simulink model "USV_SAR_MovingTarget"  (R2026b)
settings: Solver=VariableStepAuto  StopTime=600
undefined symbols (not defined in the file): arrival_dwell_time, arrival_radius, arrival_speed, assistance_duration, current_bias_x, current_bias_y, current_change_time, current_estimation_tau, current_x, drag_r, drag_u, F_max, home_x, home_y, inertia_z, initial_heading, initial_x, initial_y, integral_activation_radius, K_aw, K_distance, Kd_heading, Ki_position, Ki_u, Kp_heading, Kp_u, M_max, mass_usv, num_waypoints, position_integral_limit, sar_detection_range, sar_drift_factor, sar_target_x, sar_target_y, u_max, waypoints
libraries: simulink x6
settings Model: Creator=pablo  LastModifiedBy=pablo

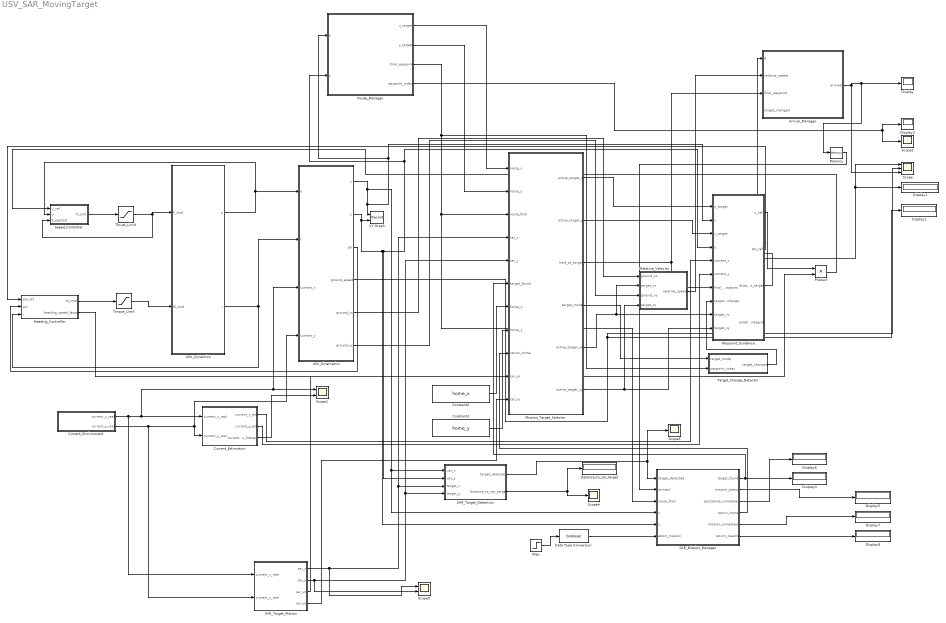
== system USV_SAR_MovingTarget ==
  Arrival_Manager : Stateflow chart  TreatAsAtomicUnit=on
  Constant2 : Constant  Value=home_x
  Constant3 : Constant  Value=home_y
  Current_Environment : Subsystem
  Current_Estimation : Subsystem
  Data Type Conversion : DataTypeConversion  OutDataTypeStr=boolean  SaturateOnIntegerOverflow=off  RndMeth=Floor
  Display{,1..8} (9 alike) : Display
  Heading_Controller : Subsystem
  Memory : Memory
  Mission_Target_Selector : Subsystem
  Product : Product
  Relative_Velocity : Subsystem
  Route_Manager : Stateflow chart  TreatAsAtomicUnit=on
  SAR_Mission_Manager : Stateflow chart  TreatAsAtomicUnit=on
  SAR_Target_Detection : Subsystem
  SAR_Target_Motion : Subsystem
  Scope : Scope  NumInputPorts=3
      settings: ActiveDisplayYMinimum=-3.9141031212329302  ActiveDisplayYMaximum=39.009126348576444
  Scope1 : Scope  NumInputPorts=2
      settings: ActiveDisplayYMinimum=-0.25  ActiveDisplayYMaximum=0.25
  Scope2 : Scope
      settings: ActiveDisplayYMinimum=-8.8280515458215767  ActiveDisplayYMaximum=9.3125380233394175  DataLoggingVariableName=ScopeData2
  Scope3 : Scope
      settings: ActiveDisplayYMinimum=0.096949603045415472  ActiveDisplayYMaximum=1.0318774717483707  DataLoggingVariableName=ScopeData3
  Scope4 : Scope
      settings: ActiveDisplayYMinimum=-1.9004946435428702E+6  ActiveDisplayYMaximum=1.5322246928084393E+6  DataLoggingVariableName=ScopeData4
  Scope5 : Scope  NumInputPorts=2
      settings: ActiveDisplayYMinimum=-44.000000000000014  ActiveDisplayYMaximum=76.000000000000028  DataLoggingVariableName=ScopeData5
  Speed_Controller : Subsystem
  Step : Step  Time=100  FinalValue=0  SampleTime=0
  Target_Change_Detector : Subsystem
  Thrust_Limit : Saturate  UpperLimit=F_max  LowerLimit=-F_max
  Torque_Limit : Saturate  UpperLimit=M_max  LowerLimit=-M_max
  USV_Dynamics : Subsystem
  USV_Kinematics : Subsystem
  Waypoint_Guidance : Subsystem
  XY Graph : Record  NumPorts=2.0  FileSettingsInternal="{\"entries\":[{\"content\":{\"excelSettings\":{\"content\":{},\"type\":\"Streamout.ExcelSettings\"},\"parquetSettings\":{\"content\":{},\"type\":\"Streamout.ParquetSettings\"}},\"type\":\"Streamout.FileSettingStorage\",\"uuid\":\"\"}],\"packageUris\":[\"http:\\/\\/schema.mathworks.com\\/mf0\\/streamout_blocks\\/R2020a\"],\"version\":\"1.0\"}"  FrameSettings=[0, 0]  Layout=[1 1]  SignalsInternal="{\"entries\":[{\"content\":{\"signals\":[{\"content\":{\"blockPath\":[],\"dimensions\":[1],\"domain\":\"\",\"lineColor\":\"#a2142f\",\"plots\":[ 1 ],\"port\":1,\"sid\":[\"\"],\"signalID\":1,\"signalName\":\"USV_Kinematics:1\"},\"type\":\"RecordBlkView.Signal\",\"uuid\":\"\"},{\"content\":{\"blockPath\":[],\"dimensions\":[1],\"domain\":\"\",\"lineColor\":\"#139fff\",\"plots\":[ 1 ],\"port\":2,\"sid\":[\"\"],\"signalID\":2,\"signalName\":\"USV_Kinematics:2\"},\"type\":\"RecordBlkView.Signal\",\"uuid\":\"\"}]},\"type\":\"RecordBlkView.InputSignals\",\"uuid\":\"\"}],\"packageUris\":[\"http:\\/\\/schema.mathworks.com\\/mf0\\/streamout_blocks\\/R2020a\"],\"version\":\"1.0\"}"  VisualizationBindings="{\"xyplotplugin\":{\"info\":[{\"series\":[{\"bindingParametersList\":[{\"parameter\":\"X-Axis\",\"signalID\":1,\"signalName\":\"USV_Kinematics:1\"},{\"parameter\":\"Y-Axis\",\"signalID\":2,\"signalName\":\"USV_Kinematics:2\"}],\"seriesID\":0},{\"bindingParametersList\":[],\"seriesID\":1}],\"subplotID\":1}]}}"  CompatibilityTag=XY
  distance_to_sar_target : Display
  wires:
  USV_Dynamics/1(u) -> Speed_Controller/2(u), USV_Kinematics/1(u)
  USV_Dynamics/2(r) -> Heading_Controller/3(r), USV_Kinematics/2(r)
  Speed_Controller/1(F_cmd) -> Thrust_Limit/1
  Heading_Controller/1(M_cmd) -> Torque_Limit/1
  USV_Kinematics/3(psi) -> Heading_Controller/2(psi)
  USV_Kinematics/1(x) -> SAR_Mission_Manager/4(x), SAR_Target_Detection/1(usv_x), XY Graph/1, Route_Manager/1(x), Waypoint_Guidance/2(x)
  USV_Kinematics/2(y) -> SAR_Mission_Manager/5(y), SAR_Target_Detection/2(usv_y), Route_Manager/2(y), Waypoint_Guidance/4(y), XY Graph/2
  Waypoint_Guidance/2(psi_ref) -> Heading_Controller/1(psi_ref)
  Waypoint_Guidance/1(u_ref) -> Product/1
  Arrival_Manager/1(arrived) -> Memory/1, Display/1, Scope/3
  Waypoint_Guidance/3(distance_to_target) -> Arrival_Manager/1(d), Scope/1, Display1/1
  Thrust_Limit/1 -> USV_Dynamics/1(F_cmd), Speed_Controller/3(F_applied)
  Torque_Limit/1 -> USV_Dynamics/2(M_cmd)
  Heading_Controller/2(heading_speed_factor) -> Product/2
  Product/1 -> Speed_Controller/1(u_ref)
  USV_Kinematics/4(ground_speed) -> Scope/2, Display2/1
  Current_Estimation/1(current_x_est) -> Waypoint_Guidance/5(current_x)
  Current_Estimation/2(current_y_est) -> Waypoint_Guidance/6(current_y)
  Current_Estimation/3(current_x_filtered) -> Scope1/2
  Current_Environment/1(current_x_real) -> SAR_Target_Motion/1(current_x_real), Scope1/1, USV_Kinematics/3(current_x), Current_Estimation/1(current_x_real)
  Current_Environment/2(current_y_real) -> SAR_Target_Motion/2(current_y_real), Current_Estimation/2(current_y_real), USV_Kinematics/4(current_y)
  Route_Manager/4(waypoint_index) -> Scope2/1, Display3/1
  SAR_Target_Motion/1(sar_x) -> Mission_Target_Selector/4(sar_x), SAR_Target_Detection/3(target_x), Scope5/1
  SAR_Target_Motion/2(sar_y) -> Mission_Target_Selector/5(sar_y), SAR_Target_Detection/4(target_y), Scope5/2
  SAR_Mission_Manager/1(target_found) -> Mission_Target_Selector/6(target_found), Display4/1
  SAR_Mission_Manager/2(mission_status) -> Display5/1
  Memory/1 -> SAR_Mission_Manager/2(arrived)
  SAR_Target_Detection/1(target_detected) -> Scope3/1, SAR_Mission_Manager/1(target_detected)
  SAR_Target_Detection/2(distance_to_sar_target) -> distance_to_sar_target/1, Scope4/1
  Mission_Target_Selector/3(hold_at_target) -> Arrival_Manager/3(final_waypoint), Waypoint_Guidance/7(final_waypoint)
  Route_Manager/1(x_target) -> Mission_Target_Selector/1(route_x)
  Route_Manager/2(y_target) -> Mission_Target_Selector/2(route_y)
  Route_Manager/3(final_waypoint) -> Target_Change_Detector/2(waypoint_index), SAR_Mission_Manager/3(route_final), Mission_Target_Selector/3(route_final)
  Mission_Target_Selector/1(active_target_x) -> Waypoint_Guidance/1(x_target)
  Mission_Target_Selector/2(active_target_y) -> Waypoint_Guidance/3(y_target)
  SAR_Mission_Manager/3(assistance_completed) -> Display6/1
  Constant2/1 -> Mission_Target_Selector/7(home_x)
  Constant3/1 -> Mission_Target_Selector/8(home_y)
  SAR_Mission_Manager/4(return_home) -> Mission_Target_Selector/9(return_home)
  SAR_Mission_Manager/5(mission_completed) -> Display7/1
  Step/1 -> Data Type Conversion/1
  Data Type Conversion/1 -> SAR_Mission_Manager/6(abort_mission)
  SAR_Mission_Manager/6(return_reason) -> Display8/1
  Target_Change_Detector/1(target_changed) -> Waypoint_Guidance/8(target_change)
  Mission_Target_Selector/4(target_mode) -> Target_Change_Detector/1(target_mode)
  SAR_Target_Motion/3(sar_vx) -> Mission_Target_Selector/10(sar_vx)
  SAR_Target_Motion/4(sar_vy) -> Mission_Target_Selector/11(sar_vy)
  Mission_Target_Selector/5(active_target_vx) -> Relative_Velocity/2(target_vx), Waypoint_Guidance/9(target_vx)
  Mission_Target_Selector/6(active_target_vy) -> Relative_Velocity/4(target_vy), Waypoint_Guidance/10(target_vy)
  USV_Kinematics/5(ground_vx) -> Relative_Velocity/1(ground_vx)
  USV_Kinematics/6(ground_vy) -> Relative_Velocity/3(ground_vy)
  Relative_Velocity/1(relative_speed) -> Arrival_Manager/2(relative_speed)

== system USV_SAR_MovingTarget/Current_Environment ==
  Step : Step  Time=current_change_time  InitialValue=current_x  FinalValue=current_x_after  SampleTime=0
  Step1 : Step  Time=current_change_time  InitialValue=current_y  FinalValue=current_y_after  SampleTime=0
  current_x_real : Outport
  current_y_real : Outport  Port=2
  wires:
  Step/1 -> current_x_real/1
  Step1/1 -> current_y_real/1

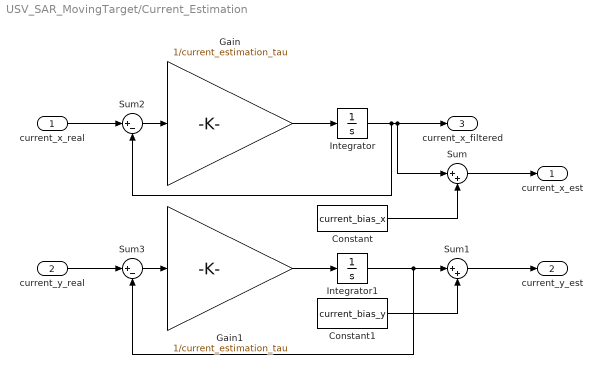
== system USV_SAR_MovingTarget/Current_Estimation ==
  current_x_real : Inport
  current_y_real : Inport  Port=2
  Constant : Constant  Value=current_bias_x
  Constant1 : Constant  Value=current_bias_y
  Gain : Gain  Gain=1/current_estimation_tau
  Gain1 : Gain  Gain=1/current_estimation_tau
  Integrator : Integrator  InitialCondition=current_x
  Integrator1 : Integrator  InitialCondition=current_x
  Sum : Sum  Inputs=|++
  Sum1 : Sum  Inputs=|++
  Sum2 : Sum  Inputs=|+-
  Sum3 : Sum  Inputs=|+-
  current_x_est : Outport
  current_y_est : Outport  Port=2
  current_x_filtered : Outport  Port=3
  wires:
  current_y_real/1 -> Sum3/1
  current_x_real/1 -> Sum2/1
  Gain1/1 -> Integrator1/1
  Sum2/1 -> Gain/1
  Sum3/1 -> Gain1/1
  Gain/1 -> Integrator/1
  Integrator/1 -> Sum/1, current_x_filtered/1, Sum2/2
  Constant/1 -> Sum/2
  Integrator1/1 -> Sum3/2, Sum1/1
  Constant1/1 -> Sum1/2
  Sum/1 -> current_x_est/1
  Sum1/1 -> current_y_est/1

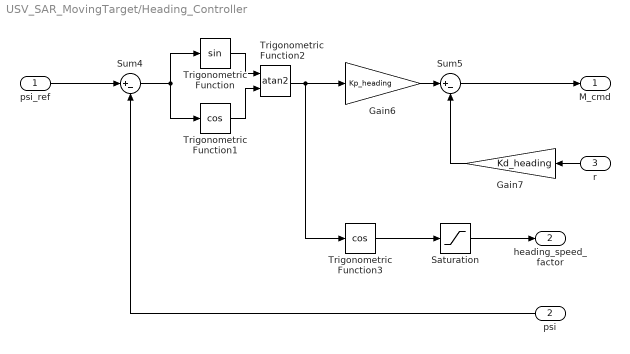
== system USV_SAR_MovingTarget/Heading_Controller ==
  psi_ref : Inport
  psi : Inport  Port=2
  r : Inport  Port=3
  Gain6 : Gain  Gain=Kp_heading
  Gain7 : Gain  Gain=Kd_heading
  Saturation : Saturate  UpperLimit=1  LowerLimit=0
  Sum4 : Sum  Inputs=|+-
  Sum5 : Sum  Inputs=|+-
  Trigonometric Function : Trigonometry
  Trigonometric Function1 : Trigonometry  Operator=cos
  Trigonometric Function2 : Trigonometry  Operator=atan2
  Trigonometric Function3 : Trigonometry  Operator=cos
  M_cmd : Outport
  heading_speed_factor : Outport  Port=2
  wires:
  Sum5/1 -> M_cmd/1
  psi_ref/1 -> Sum4/1
  r/1 -> Gain7/1
  Gain6/1 -> Sum5/1
  psi/1 -> Sum4/2
  Gain7/1 -> Sum5/2
  Sum4/1 -> Trigonometric Function/1, Trigonometric Function1/1
  Trigonometric Function/1 -> Trigonometric Function2/1
  Trigonometric Function1/1 -> Trigonometric Function2/2
  Trigonometric Function2/1 -> Trigonometric Function3/1, Gain6/1
  Trigonometric Function3/1 -> Saturation/1
  Saturation/1 -> heading_speed_factor/1

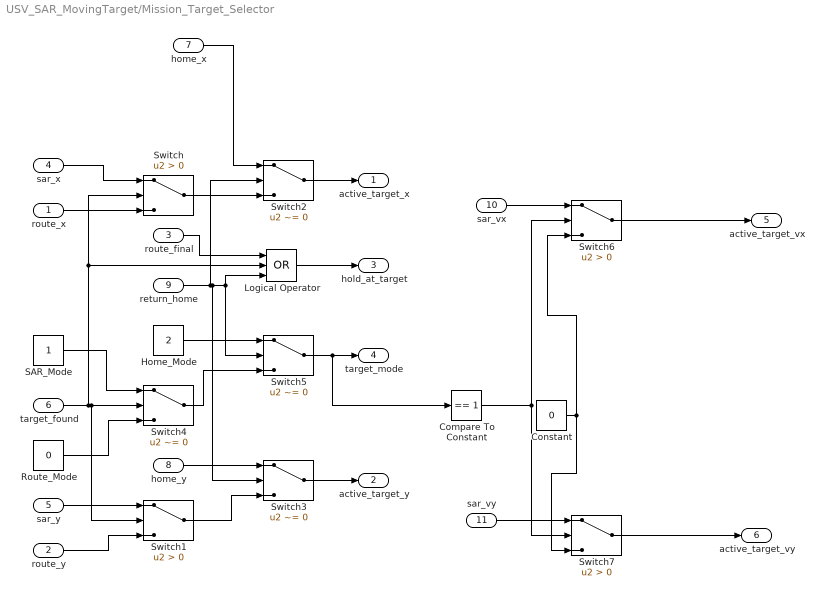
== system USV_SAR_MovingTarget/Mission_Target_Selector ==
  route_x : Inport
  route_y : Inport  Port=2
  route_final : Inport  Port=3
  sar_x : Inport  Port=4
  sar_y : Inport  Port=5
  target_found : Inport  Port=6
  home_x : Inport  Port=7
  home_y : Inport  Port=8
  return_home : Inport  Port=9
  sar_vx : Inport  Port=10
  sar_vy : Inport  Port=11
  Compare To Constant : simulink/Logic and Bit Operations/Compare To Constant  relop===  const=1  OutDataTypeStr=boolean
  Constant : Constant  Value=0
  Home_Mode : Constant  Value=2
  Logical Operator : Logic  Operator=OR  Inputs=3  AllPortsSameDT=off  OutDataTypeStr=boolean
  Route_Mode : Constant  Value=0
  SAR_Mode : Constant
  Switch{,1,6..7} (4 alike) : Switch  Criteria=u2 > Threshold  SaturateOnIntegerOverflow=off  InputSameDT=off
  Switch{2..5} (4 alike) : Switch  Criteria=u2 ~= 0  SaturateOnIntegerOverflow=off  InputSameDT=off
  active_target_x : Outport
  active_target_y : Outport  Port=2
  hold_at_target : Outport  Port=3
  target_mode : Outport  Port=4
  active_target_vx : Outport  Port=5
  active_target_vy : Outport  Port=6
  wires:
  route_final/1 -> Logical Operator/1
  home_x/1 -> Switch2/1
  target_found/1 -> Switch1/2, Switch4/2, Logical Operator/2, Switch/2
  route_y/1 -> Switch1/3
  route_x/1 -> Switch/3
  sar_y/1 -> Switch1/1
  home_y/1 -> Switch3/1
  sar_x/1 -> Switch/1
  Switch4/1 -> Switch5/3
  Route_Mode/1 -> Switch4/3
  SAR_Mode/1 -> Switch4/1
  Switch/1 -> Switch2/3
  return_home/1 -> Logical Operator/3, Switch5/2, Switch3/2, Switch2/2
  Home_Mode/1 -> Switch5/1
  Switch1/1 -> Switch3/3
  Logical Operator/1 -> hold_at_target/1
  Switch2/1 -> active_target_x/1
  Switch5/1 -> Compare To Constant/1, target_mode/1
  Switch3/1 -> active_target_y/1
  Compare To Constant/1 -> Switch6/2, Switch7/2
  sar_vx/1 -> Switch6/1
  sar_vy/1 -> Switch7/1
  Constant/1 -> Switch7/3, Switch6/3
  Switch6/1 -> active_target_vx/1
  Switch7/1 -> active_target_vy/1

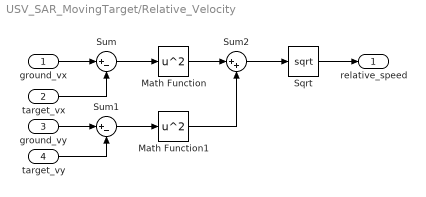
== system USV_SAR_MovingTarget/Relative_Velocity ==
  ground_vx : Inport
  target_vx : Inport  Port=2
  ground_vy : Inport  Port=3
  target_vy : Inport  Port=4
  Math Function : Math  Operator=square
  Math Function1 : Math  Operator=square
  Sqrt : Sqrt
  Sum : Sum  Inputs=|+-
  Sum1 : Sum  Inputs=|+-
  Sum2 : Sum  Inputs=|++
  relative_speed : Outport
  wires:
  Sum/1 -> Math Function/1
  ground_vx/1 -> Sum/1
  Math Function1/1 -> Sum2/2
  target_vx/1 -> Sum/2
  ground_vy/1 -> Sum1/1
  Math Function/1 -> Sum2/1
  target_vy/1 -> Sum1/2
  Sum1/1 -> Math Function1/1
  Sum2/1 -> Sqrt/1
  Sqrt/1 -> relative_speed/1

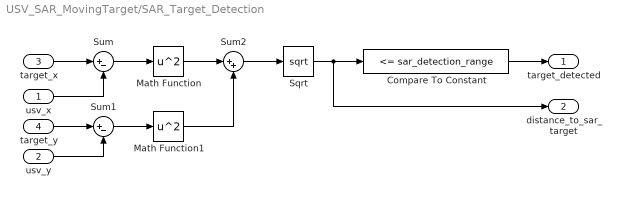
== system USV_SAR_MovingTarget/SAR_Target_Detection ==
  usv_x : Inport
  usv_y : Inport  Port=2
  target_x : Inport  Port=3
  target_y : Inport  Port=4
  Compare To Constant : simulink/Logic and Bit Operations/Compare To Constant  relop=<=  const=sar_detection_range  OutDataTypeStr=boolean
  Math Function : Math  Operator=square
  Math Function1 : Math  Operator=square
  Sqrt : Sqrt
  Sum : Sum  Inputs=|+-
  Sum1 : Sum  Inputs=|+-
  Sum2 : Sum  Inputs=|++
  target_detected : Outport
  distance_to_sar_target : Outport  Port=2
  wires:
  Sum1/1 -> Math Function1/1
  Sum/1 -> Math Function/1
  usv_x/1 -> Sum/2
  target_x/1 -> Sum/1
  usv_y/1 -> Sum1/2
  Math Function1/1 -> Sum2/2
  Math Function/1 -> Sum2/1
  Sum2/1 -> Sqrt/1
  target_y/1 -> Sum1/1
  Sqrt/1 -> Compare To Constant/1, distance_to_sar_target/1
  Compare To Constant/1 -> target_detected/1

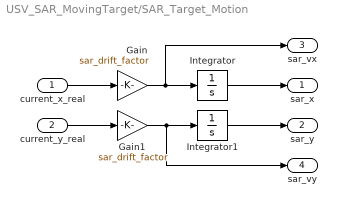
== system USV_SAR_MovingTarget/SAR_Target_Motion ==
  current_x_real : Inport
  current_y_real : Inport  Port=2
  Gain : Gain  Gain=sar_drift_factor
  Gain1 : Gain  Gain=sar_drift_factor
  Integrator : Integrator  InitialCondition=sar_target_x
  Integrator1 : Integrator  InitialCondition=sar_target_y
  sar_x : Outport
  sar_y : Outport  Port=2
  sar_vx : Outport  Port=3
  sar_vy : Outport  Port=4
  wires:
  current_y_real/1 -> Gain1/1
  current_x_real/1 -> Gain/1
  Gain/1 -> sar_vx/1, Integrator/1
  Gain1/1 -> sar_vy/1, Integrator1/1
  Integrator/1 -> sar_x/1
  Integrator1/1 -> sar_y/1

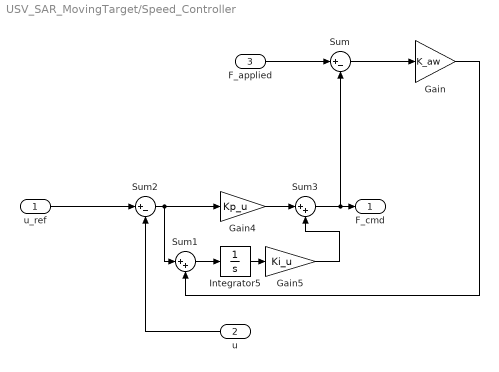
== system USV_SAR_MovingTarget/Speed_Controller ==
  u_ref : Inport
  u : Inport  Port=2
  F_applied : Inport  Port=3
  Gain : Gain  Gain=K_aw
  Gain4 : Gain  Gain=Kp_u
  Gain5 : Gain  Gain=Ki_u
  Integrator5 : Integrator
  Sum : Sum  Inputs=|+-
  Sum1 : Sum  Inputs=|++
  Sum2 : Sum  Inputs=|+-
  Sum3 : Sum  Inputs=|++
  F_cmd : Outport
  wires:
  Integrator5/1 -> Gain5/1
  u_ref/1 -> Sum2/1
  u/1 -> Sum2/2
  Gain5/1 -> Sum3/2
  Sum2/1 -> Sum1/1, Gain4/1
  Gain4/1 -> Sum3/1
  Sum3/1 -> Sum/2, F_cmd/1
  F_applied/1 -> Sum/1
  Sum/1 -> Gain/1
  Sum1/1 -> Integrator5/1
  Gain/1 -> Sum1/2

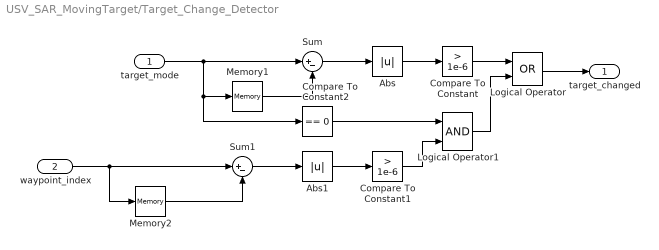
== system USV_SAR_MovingTarget/Target_Change_Detector ==
  target_mode : Inport
  waypoint_index : Inport  Port=2
  Abs : Abs  SaturateOnIntegerOverflow=off
  Abs1 : Abs  SaturateOnIntegerOverflow=off
  Compare To Constant : simulink/Logic and Bit Operations/Compare To Constant  relop=>  const=1e-6  OutDataTypeStr=boolean
  Compare To Constant1 : simulink/Logic and Bit Operations/Compare To Constant  relop=>  const=1e-6  OutDataTypeStr=boolean
  Compare To Constant2 : simulink/Logic and Bit Operations/Compare To Constant  relop===  const=0  OutDataTypeStr=boolean
  Logical Operator : Logic  Operator=OR  AllPortsSameDT=off  OutDataTypeStr=boolean
  Logical Operator1 : Logic  AllPortsSameDT=off  OutDataTypeStr=boolean
  Memory1 : Memory
  Memory2 : Memory  InitialCondition=1
  Sum : Sum  Inputs=|+-
  Sum1 : Sum  Inputs=|+-
  target_changed : Outport
  wires:
  target_mode/1 -> Compare To Constant2/1, Memory1/1, Sum/1
  Abs1/1 -> Compare To Constant1/1
  waypoint_index/1 -> Sum1/1, Memory2/1
  Sum/1 -> Abs/1
  Memory2/1 -> Sum1/2
  Sum1/1 -> Abs1/1
  Memory1/1 -> Sum/2
  Compare To Constant2/1 -> Logical Operator1/1
  Abs/1 -> Compare To Constant/1
  Logical Operator1/1 -> Logical Operator/2
  Compare To Constant1/1 -> Logical Operator1/2
  Compare To Constant/1 -> Logical Operator/1
  Logical Operator/1 -> target_changed/1

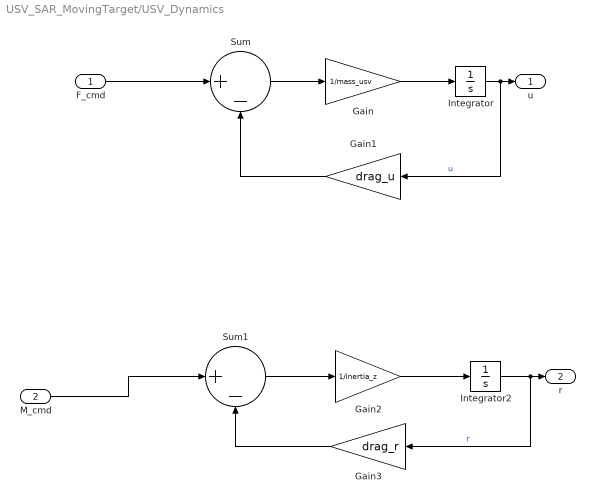
== system USV_SAR_MovingTarget/USV_Dynamics ==
  F_cmd : Inport
  M_cmd : Inport  Port=2
  Gain : Gain  Gain=1/mass_usv
  Gain1 : Gain  Gain=drag_u
  Gain2 : Gain  Gain=1/inertia_z
  Gain3 : Gain  Gain=drag_r
  Integrator : Integrator
  Integrator2 : Integrator
  Sum : Sum  Inputs=|+-
  Sum1 : Sum  Inputs=|+-
  u : Outport
  r : Outport  Port=2
  wires:
  F_cmd/1 -> Sum/1
  Gain2/1 -> Integrator2/1
  Gain3/1 -> Sum1/2
  Integrator/1 -> Gain1/1, u/1  "u"
  Sum/1 -> Gain/1
  Gain/1 -> Integrator/1
  Gain1/1 -> Sum/2
  Sum1/1 -> Gain2/1
  Integrator2/1 -> Gain3/1, r/1  "r"
  M_cmd/1 -> Sum1/1

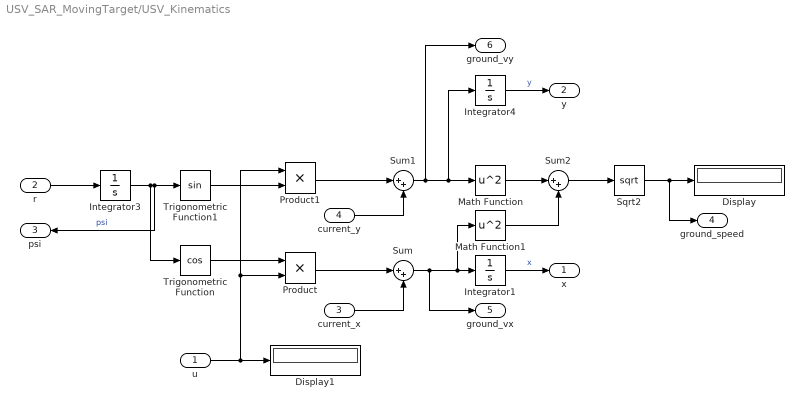
== system USV_SAR_MovingTarget/USV_Kinematics ==
  u : Inport
  r : Inport  Port=2
  current_x : Inport  Port=3
  current_y : Inport  Port=4
  Display : Display
  Display1 : Display
  Integrator1 : Integrator  InitialCondition=initial_x
  Integrator3 : Integrator  InitialCondition=initial_heading
  Integrator4 : Integrator  InitialCondition=initial_y
  Math Function : Math  Operator=square
  Math Function1 : Math  Operator=square
  Product : Product
  Product1 : Product
  Sqrt2 : Sqrt
  Sum : Sum  Inputs=|++
  Sum1 : Sum  Inputs=|++
  Sum2 : Sum  Inputs=|++
  Trigonometric Function : Trigonometry  Operator=cos
  Trigonometric Function1 : Trigonometry
  x : Outport
  y : Outport  Port=2
  psi : Outport  Port=3
  ground_speed : Outport  Port=4
  ground_vx : Outport  Port=5
  ground_vy : Outport  Port=6
  wires:
  Math Function/1 -> Sum2/1
  current_y/1 -> Sum1/2
  Integrator3/1 -> psi/1, Trigonometric Function1/1, Trigonometric Function/1  "psi"
  u/1 -> Product/2, Product1/1, Display1/1
  r/1 -> Integrator3/1
  Product/1 -> Sum/1
  Math Function1/1 -> Sum2/2
  Product1/1 -> Sum1/1
  Trigonometric Function/1 -> Product/1
  Trigonometric Function1/1 -> Product1/2
  current_x/1 -> Sum/2
  Sqrt2/1 -> Display/1, ground_speed/1
  Sum1/1 -> ground_vy/1, Math Function/1, Integrator4/1
  Sum2/1 -> Sqrt2/1
  Sum/1 -> ground_vx/1, Math Function1/1, Integrator1/1
  Integrator4/1 -> y/1  "y"
  Integrator1/1 -> x/1  "x"

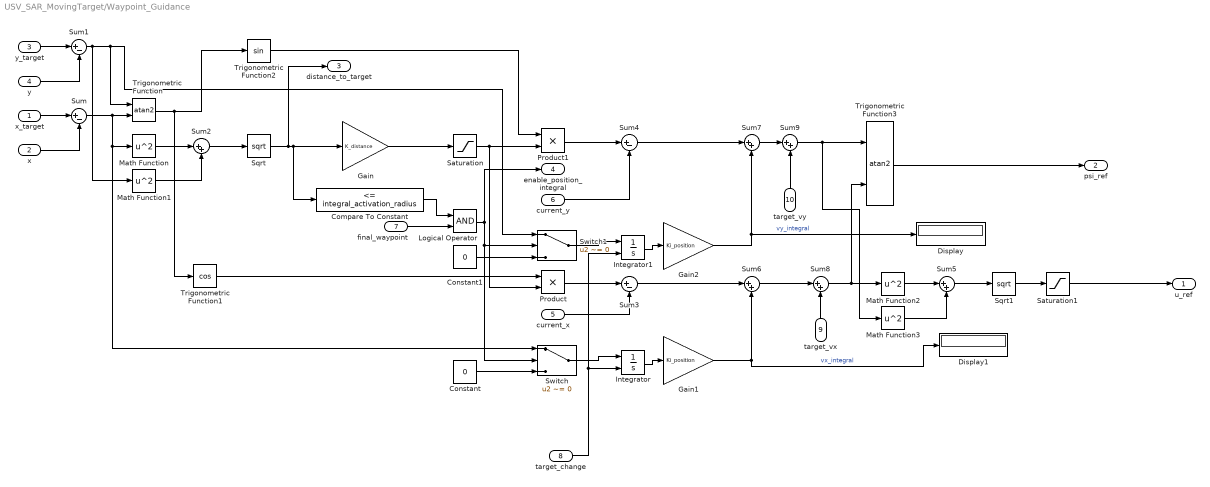
== system USV_SAR_MovingTarget/Waypoint_Guidance ==
  x_target : Inport
  x : Inport  Port=2
  y_target : Inport  Port=3
  y : Inport  Port=4
  current_x : Inport  Port=5
  current_y : Inport  Port=6
  final_waypoint : Inport  Port=7
  target_change : Inport  Port=8
  target_vx : Inport  Port=9
  target_vy : Inport  Port=10
  Compare To Constant : simulink/Logic and Bit Operations/Compare To Constant  relop=<=  const=integral_activation_radius  OutDataTypeStr=boolean
  Constant : Constant  Value=0
  Constant1 : Constant  Value=0
  Display : Display
  Display1 : Display
  Gain : Gain  Gain=K_distance
  Gain1 : Gain  Gain=Ki_position
  Gain2 : Gain  Gain=Ki_position
  Integrator : Integrator  ExternalReset=rising  LimitOutput=on  UpperSaturationLimit=position_integral_limit  LowerSaturationLimit=-position_integral_limit
  Integrator1 : Integrator  ExternalReset=rising  LimitOutput=on  UpperSaturationLimit=position_integral_limit  LowerSaturationLimit=-position_integral_limit
  Logical Operator : Logic  AllPortsSameDT=off  OutDataTypeStr=boolean
  Math Function{,1..3} (4 alike) : Math  Operator=square
  Product : Product
  Product1 : Product
  Saturation : Saturate  UpperLimit=u_max  LowerLimit=0
  Saturation1 : Saturate  UpperLimit=u_max  LowerLimit=0
  Sqrt : Sqrt
  Sqrt1 : Sqrt
  Sum{,1,3..4} (4 alike) : Sum  Inputs=|+-
  Sum{2,5..9} (6 alike) : Sum  Inputs=|++
  Switch : Switch  Criteria=u2 ~= 0  SaturateOnIntegerOverflow=off  InputSameDT=off
  Switch1 : Switch  Criteria=u2 ~= 0  SaturateOnIntegerOverflow=off  InputSameDT=off
  Trigonometric Function : Trigonometry  Operator=atan2
  Trigonometric Function1 : Trigonometry  Operator=cos
  Trigonometric Function2 : Trigonometry
  Trigonometric Function3 : Trigonometry  Operator=atan2
  u_ref : Outport
  psi_ref : Outport  Port=2
  distance_to_target : Outport  Port=3
  enable_position_integral : Outport  Port=4
  wires:
  Product/1 -> Sum3/1
  current_y/1 -> Sum4/2
  x/1 -> Sum/2
  x_target/1 -> Sum/1
  Product1/1 -> Sum4/1
  y/1 -> Sum1/2
  y_target/1 -> Sum1/1
  Switch1/1 -> Integrator1/1
  Trigonometric Function/1 -> Trigonometric Function2/1, Trigonometric Function1/1
  Math Function/1 -> Sum2/1
  Math Function2/1 -> Sum5/1
  Sum2/1 -> Sqrt/1
  Sum/1 -> Switch/1, Math Function/1, Trigonometric Function/2
  Sqrt/1 -> Gain/1, Compare To Constant/1, distance_to_target/1
  Sum1/1 -> Switch1/1, Trigonometric Function/1, Math Function1/1
  Saturation1/1 -> u_ref/1
  Math Function1/1 -> Sum2/2
  Trigonometric Function1/1 -> Product/1
  Switch/1 -> Integrator/1
  Trigonometric Function2/1 -> Product1/1
  Gain/1 -> Saturation/1
  Compare To Constant/1 -> Logical Operator/1
  final_waypoint/1 -> Logical Operator/2
  Constant/1 -> Switch/3
  Saturation/1 -> Product/2, Product1/2
  Sum4/1 -> Sum7/1
  Logical Operator/1 -> Switch/2, Switch1/2, enable_position_integral/1
  Constant1/1 -> Switch1/3
  current_x/1 -> Sum3/2
  Integrator1/1 -> Gain2/1
  Sum3/1 -> Sum6/1
  Integrator/1 -> Gain1/1
  Gain2/1 -> Sum7/2, Display/1  "vy_integral"
  Gain1/1 -> Sum6/2, Display1/1  "vx_integral"
  Trigonometric Function3/1 -> psi_ref/1
  Sum5/1 -> Sqrt1/1
  Math Function3/1 -> Sum5/2
  Sqrt1/1 -> Saturation1/1
  target_change/1 -> Integrator/2, Integrator1/2
  Sum6/1 -> Sum8/1
  Sum8/1 -> Math Function2/1, Trigonometric Function3/2
  target_vx/1 -> Sum8/2
  Sum7/1 -> Sum9/1
  Sum9/1 -> Math Function3/1, Trigonometric Function3/1
  target_vy/1 -> Sum9/2

== stateflow chart USV_SAR_MovingTarget/Route_Manager ==
  state Following_Route
    entry:
    waypoint_index = 1;
    x_target = waypoints(waypoint_index, 1);
    y_target = waypoints(waypoint_index, 2);
    final_waypoint = (waypoint_index == num_waypoints);
    during:
    if waypoint_index < num_waypoints && ...
    (x_target-x)^2 + (y_target-y)^2 <= arrival_radius^2
    waypoint_index = waypoint_index + 1;
    end
    x_target = waypoints(waypoint_index, 1);
    y_target = waypoints(waypoint_index, 2);
    final_waypoint = (waypoint_index == num_waypoints);
  (default) -> Following_Route
  data: x input; y input; x_target output; y_target output; final_waypoint output; arrival_radius parameter; waypoints parameter; num_waypoints parameter size=1; waypoint_index output size=1

== stateflow chart USV_SAR_MovingTarget/SAR_Mission_Manager ==
  state Searching
    entry:
    target_found = false;
    mission_status = 0;
    assistance_completed = false;
    return_home=false;
    mission_completed=false;
    return_reason=0;
  state Approaching
    entry:
    target_found = true;
    mission_status = 1;
  state Search_Completed
    entry:
    target_found = false;
    mission_status = 3;
  state On_Scene
    entry:
    target_found = true;
    mission_status = 2;
    during:
    if ~abort_mission && after(assistance_duration,sec)
    assistance_completed=true;
    end
  state Home_Reached
    entry:
    return_home=true;
    mission_status=5;
    mission_completed=true;
  state Returning_Home
    entry:
    return_home=true;
    mission_status=4;
    if abort_mission
    return_reason=3;
    elseif assistance_completed
    return_reason=1;
    else
    return_reason=2;
    end
  (default) -> Searching
  Searching -> Returning_Home [order 2] : [abort_mission]
  Searching -> Search_Completed [order 3] : [route_final == 1 && arrived == 1 && ~target_detected]
  Searching -> Approaching [order 1] : [~abort_mission && target_detected]
  Search_Completed -> Approaching [order 1] : [~abort_mission && target_detected]
  Approaching -> Returning_Home [order 2] : [abort_mission]
  On_Scene -> Approaching [order 1] : [arrived == 0]
  Approaching -> On_Scene [order 1] : [~abort_mission && arrived==1]
  Search_Completed -> Returning_Home [order 2] : [abort_mission || ~target_detected]
  On_Scene -> Returning_Home [order 2] : [~abort_mission && assistance_completed && arrived==1]
  Returning_Home -> Home_Reached : [arrived==1 && (x-home_x)^2+(y-home_y)^2 <= arrival_radius^2]
  On_Scene -> Returning_Home [order 3] : [abort_mission]
  data: target_detected input boolean; target_found output boolean; arrived input; mission_status output; route_final input; assistance_duration parameter; assistance_completed output; return_home output; x input; y input; home_x parameter; home_y parameter; arrival_radius parameter; mission_completed output; abort_mission input; return_reason output

== stateflow chart USV_SAR_MovingTarget/Arrival_Manager ==
  state Navigating
    entry:
    arrived = 0;
  state Settling
    entry:
    arrived = 0;
  state Confirming
    entry:
    arrived = 0;
  state Arrived
    entry:
    arrived = 1;
  (default) -> Navigating
  Confirming -> Navigating [order 3] : [final_waypoint == 0||target_changed]
  Arrived -> Navigating [order 2] : [target_changed]
  Settling -> Navigating [order 2] : [final_waypoint == 0||target_changed]
  Navigating -> Settling : [~target_changed && final_waypoint==1 && d<=arrival_radius]
  Arrived -> Settling [order 1] : [d > 2*arrival_radius || relative_speed > 2*arrival_speed]
  Confirming -> Settling [order 1] : [d > arrival_radius || relative_speed > arrival_speed]
  Settling -> Confirming [order 1] : [d <= arrival_radius && relative_speed <= arrival_speed]
  Confirming -> Arrived [order 2] : [after(arrival_dwell_time, sec) && d <= arrival_radius && relative_speed <= arrival_speed]
  data: d input; relative_speed input; arrived output; final_waypoint input; arrival_speed parameter; arrival_radius parameter; arrival_dwell_time parameter; target_changed input
